simulink library "SignalSourceBlockLibrary"  (R2023a)
settings: Solver=VariableStepAuto  StartTime=0.0  StopTime=10.0  RelTol=1e-3
libraries: simulink x4
settings Model: Creator=isaacito  LastModifiedBy=isaacito
settings OptimizationCC: ReuseModelBlockBuffer=off

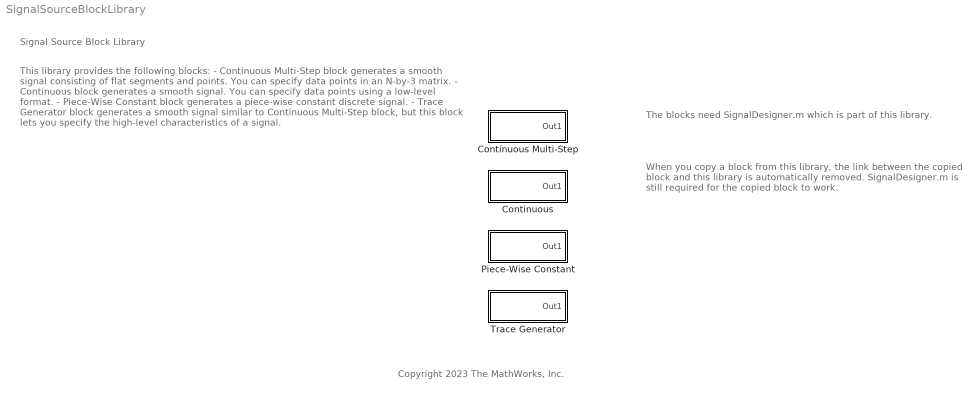
== system SignalSourceBlockLibrary ==
  note: The blocks need SignalDesigner.m
      | which is part of this library.
  note: When you copy a block from this library,
      | the link between the copied block and
      | this library is automatically removed.
      | SignalDesigner.m is still required for
      | the copied block to work.
  note: Copyright 2023 The MathWorks, Inc.
  note: Signal Source Block Library
  note: This library provides the following blocks:
      |
      | - Continuous Multi-Step block generates
      | a smooth signal consisting of flat segments and points.
      | You can specify data points in an N-by-3 matrix.
      |
      | - Continuous block generates a smooth signal.
      | You can specify data points using a low-level format.
      |
      | - Piece-Wise Constant block generates
      | a piece-wise constant discrete signal.
      |
      | - Trace Generator block generates a smooth signal
      | similar to Continuous Multi-Step block, but
      | this block lets you specify the high-level characteristics
      | of a signal.
  Continuous : Subsystem  mask(Continuous Multi-Step Signal){dataPoints=[0 0; 1 0; 2 5; 4 2; 5 2], deltaT=0.05}
      mask prompts: dataPoints "Data points"; deltaT "Interpolation step [s]"
      mask help:
      | This block generates a signal consisting of smoothly connected flat segments. Data points parameter takes an N-by-3 matrix where each row specifies a flat segment. First column and second column define start and end time of the segment, respectively. Third column defines the value of the segment. Second column can also be NaN to define a point value. Flat segments and point values are smoothly interpolated by Akima spline with the specified interpolation step.
      |
      | For example, a matrix [0 1 5; 3 nan 9; 6 8 7] for Data points defines a signal as follows. First row defines a flat segment from t=0 to t=1 of value 5. Second row defines a point at t=3 of value 9. Third row defines a flat segment from t=6 to t=8 of value 7.
      mask init:
      | sig = SignalDesigner("Continuous");
      | 
      | % Initialization function can access parameter names directly
      | sig.XYData = dataPoints;
      | sig.DeltaX = deltaT;
      | 
      | update(sig)
      settings: CopyFcn=|
      | set_param(gcb, LinkStatus = "none");
      | set_param(gcb, CopyFcn = "");
      mask DialogControl Control3 Prompt: horizontal spacer 1
      mask DialogControl Control4 Prompt: horizontal spacer 2
      mask DialogControl Control5 Prompt: horizontal spacer 3
      mask DialogControl PlotButton Prompt: Plot
      mask DialogControl PlotButton Callback: SignalSourceBlockCallback.plotContinuous(gcb);
      mask Display: disp("Continuous")
  Continuous Multi-Step : Subsystem  mask(Continuous Multi-Step Signal){dataPoints=[0 1 0; 3 nan 9; 6 8 7], deltaT=0.05}
      mask prompts: dataPoints "Data points"; deltaT "Interpolation step [s]"
      mask help:
      | This block generates a signal consisting of smoothly connected flat segments. Data points parameter takes an N-by-3 matrix where each row specifies a flat segment. First column and second column define start and end time of the segment, respectively. Third column defines the value of the segment. Second column can also be NaN to define a point value. Flat segments and point values are smoothly interpolated by Akima spline with the specified interpolation step.
      |
      | For example, a matrix [0 1 5; 3 nan 9; 6 8 7] for Data points defines a signal as follows. First row defines a flat segment from t=0 to t=1 of value 5. Second row defines a point at t=3 of value 9. Third row defines a flat segment from t=6 to t=8 of value 7.
      mask init:
      | sig = SignalDesigner("ContinuousMultiStep");
      | 
      | % Initialization function can access parameter names directly
      | sig.XYData = dataPoints;
      | sig.DeltaX = deltaT;
      | 
      | update(sig)
      settings: CopyFcn=|
      | set_param(gcb, LinkStatus = "none");
      | set_param(gcb, CopyFcn = "");
      mask DialogControl Control3 Prompt: horizontal spacer 1
      mask DialogControl Control4 Prompt: horizontal spacer 2
      mask DialogControl Control5 Prompt: horizontal spacer 3
      mask DialogControl PlotButton Prompt: Plot
      mask DialogControl PlotButton Callback: SignalSourceBlockCallback.plotContinuousMultiStep(gcb);
      mask Display: disp("Continuous" + newline + "Multi-Step")
  Piece-Wise Constant : Subsystem  mask(Piece-Wise Constant Signal){dataPoints=[0 1; 2 3; 4 2; 5 2]}
      mask prompts: dataPoints "Data points"
      mask help:
      | This block generates a piece-wise constant signal. Data points parameter takes an N-by-2 matrix where each row specifies a constant segment. First column defines the start time of constant segment, and second column specifies the value of it. The value continues until the value of the next segment is defined. The values of the two consecutive rows are connected with a discrete jump.
      |
      | For example, a matrix [0 6; 1 7;2 5] for Data points defines a signal as follows. First row defines a constant segment from t=0 of value 6. Second row defines a point at t=1 of value 7. Third row defines a constant segment from t=2 of value 5. The value makes a discrete jump from one segment to the next.
      mask init:
      | sig = SignalDesigner("PieceWiseConstant");
      | 
      | % Initialization function can access parameter names directly
      | sig.XYData = dataPoints;
      | 
      | update(sig)
      settings: CopyFcn=|
      | set_param(gcb, LinkStatus = "none");
      | set_param(gcb, CopyFcn = "");
      mask DialogControl Control3 Prompt: invisible horizontal spacer 1
      mask DialogControl Control4 Prompt: invisible horizontal spacer 2
      mask DialogControl Control5 Prompt: invisible horizontal spacer 3
      mask DialogControl PlotButton Prompt: Plot
      mask DialogControl PlotButton Callback: SignalSourceBlockCallback.plotPieceWiseConstant(gcb)
      mask Display: disp("Piece-Wise" + newline + "Constant")
  Trace Generator : Subsystem  mask(Trace Generator){yScale=1, tScale=1, randomSeed=5, interpolationStepSize=0.1, tInitialFlatLength=3, yInitialValue=0, numTransitions=2, transitionRange=[2 5], flatRange=[5 10], yRange=[-5 10], tFinalTransitionDuration=3, tFinalFlatDuration=4, yFinalValue=0}
      mask prompts: yScale "Data value scaler"; tScale "Time scaler"; randomSeed "Random seed"; interpolationStepSize "Interpolation step [s]"; tInitialFlatLength "Initial constant duration"; yInitialValue "Initial data value"; numTransitions "Number of transitions"; transitionRange "Range of transition duration"; flatRange "Range of constant duration"; yRange "Range of data value"; tFinalTransitionDuration "Final transition duration"; tFinalFlatDuration "Final constant duration"; yFinalValue "Final data value"
      mask help: This block generates a smooth signal consisting of flat segments.
      mask init:
      | xydata = SignalDesignUtility.buildXYData( ...
      |   RandomSeed = randomSeed, ...
      |   XScale = tScale, ...
      |   YScale = yScale, ...
      |   XInitialFlatLength = tInitialFlatLength, ...
      |   YInitialValue = yInitialValue, ...
      |   NumTransitions  = numTransitions, ...
      |   TransitionRange = transitionRange, ...
      |   FlatRange = flatRange, ...
      |   YRange = yRange, ...
      |   XFinalTransitionLength = tFinalTransitionDuration, ...
      |   XFinalFlatLength = tFinalFlatDuration, ...
      |   YFinalValue = yFinalValue );
      | 
      | sig = SignalDesigner("ContinuousMultiStep");
      | sig.XYData = xydata;
      | sig.DeltaX = interpolationStepSize;
      | 
      | update(sig)
      settings: CopyFcn=|
      | set_param(gcb, LinkStatus = "none");
      | set_param(gcb, CopyFcn = "");
      mask DialogControl Container3 Prompt: Advanced
      mask DialogControl Control3 Prompt: horizontal spacer 1
      mask DialogControl Control4 Prompt: horizontal spacer 2
      mask DialogControl Control5 Prompt: horizontal spacer 3
      mask DialogControl PlotButton Prompt: Plot
      mask DialogControl PlotButton Callback: SignalSourceBlockCallback.plotTraceGenerator(gcb);
      mask Display: disp("Trace" + newline + "Generator")

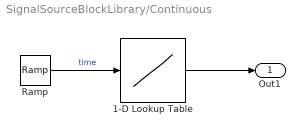
== system SignalSourceBlockLibrary/Continuous ==
  1-D Lookup Table : Lookup_n-D  NumberOfTableDimensions=1  BreakpointsForDimension1=sig.Data.X  Table=sig.Data.Y  ExtrapMethod=Clip  UseLastTableValue=on  InternalRulePriority=Speed  RndMeth=Simplest
  Ramp : simulink/Sources/Ramp  slope=1  start=0  InitialOutput=0
      settings: AttributesFormatString=|
      | Slope: %<slope>
      | Start time: %<start>
      | Initial output: %<InitialOutput>
  Out1 : Outport
  wires:
  1-D Lookup Table/1 -> Out1/1
  Ramp/1 -> 1-D Lookup Table/1  "time"

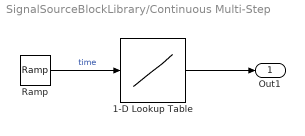
== system SignalSourceBlockLibrary/Continuous Multi-Step ==
  1-D Lookup Table : Lookup_n-D  NumberOfTableDimensions=1  BreakpointsForDimension1=sig.Data.X  Table=sig.Data.Y  InternalRulePriority=Speed  RndMeth=Simplest
  Ramp : simulink/Sources/Ramp  slope=1  start=0  InitialOutput=0
      settings: AttributesFormatString=|
      | Slope: %<slope>
      | Start time: %<start>
      | Initial output: %<InitialOutput>
  Out1 : Outport
  wires:
  1-D Lookup Table/1 -> Out1/1
  Ramp/1 -> 1-D Lookup Table/1  "time"

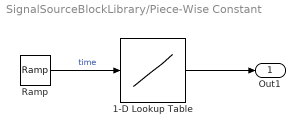
== system SignalSourceBlockLibrary/Piece-Wise Constant ==
  1-D Lookup Table : Lookup_n-D  NumberOfTableDimensions=1  BreakpointsForDimension1=sig.Data.X  Table=sig.Data.Y  InterpMethod=Flat  InternalRulePriority=Speed  RndMeth=Simplest
  Ramp : simulink/Sources/Ramp  slope=1  start=0  InitialOutput=0
      settings: AttributesFormatString=|
      | Slope: %<slope>
      | Start time: %<start>
      | Initial output: %<InitialOutput>
  Out1 : Outport
  wires:
  1-D Lookup Table/1 -> Out1/1
  Ramp/1 -> 1-D Lookup Table/1  "time"

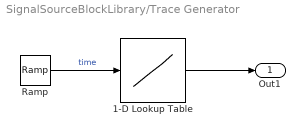
== system SignalSourceBlockLibrary/Trace Generator ==
  1-D Lookup Table : Lookup_n-D  NumberOfTableDimensions=1  BreakpointsForDimension1=sig.Data.X  Table=sig.Data.Y  InternalRulePriority=Speed  RndMeth=Simplest
  Ramp : simulink/Sources/Ramp  slope=1  start=0  InitialOutput=0
      settings: AttributesFormatString=|
      | Slope: %<slope>
      | Start time: %<start>
      | Initial output: %<InitialOutput>
  Out1 : Outport
  wires:
  Ramp/1 -> 1-D Lookup Table/1  "time"
  1-D Lookup Table/1 -> Out1/1
